simulink model "Hydrokinetic_Energy_Harvesting_Model"  (R2023a)
settings: Solver=VariableStepAuto  StartTime=0.0  StopTime=3600  RelTol=1e-3
settings Model: Creator=eeelab47  LastModifiedBy=eeelab47

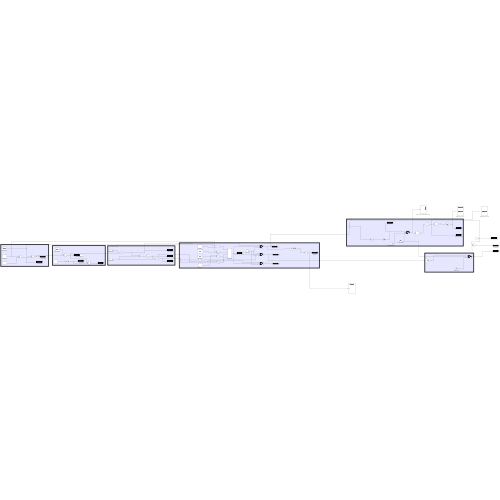
[thumbnail: Simulink's stored preview of the top-level diagram]
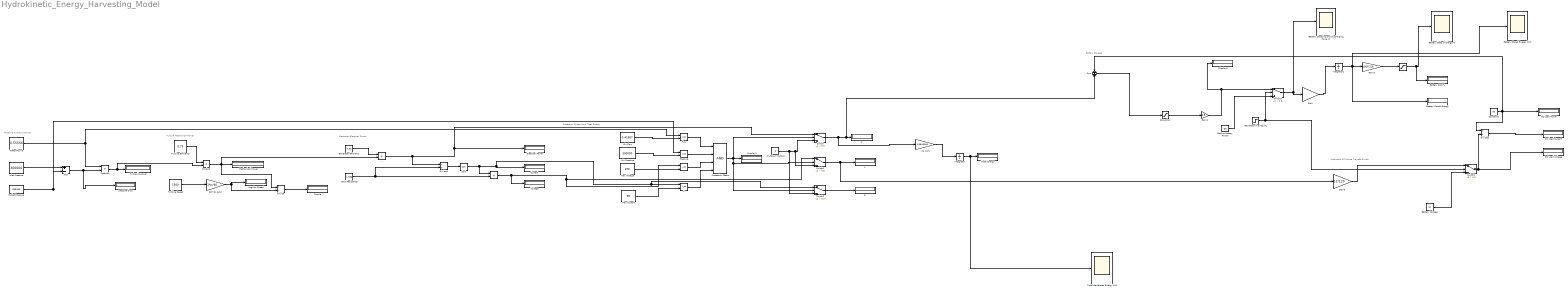
== system Hydrokinetic_Energy_Harvesting_Model ==
  note: Automatic DC Source Transfer Switch
  note: Battery Storage
  note: Protection System and Total Energy
  note: Generator Electrical Power
  note: Turbine Mechanical Power
  note: Pipeline Hydraulic Power
  " ...." : Product
  . : Saturate  UpperLimit=100  LowerLimit=0
  .. : Product
  Add : Sum  Inputs=+-
  Angular Speed : Display
  Backup Battery Power : Constant  Value=-30
  Battery Charging and Discharging Powe W : Scope
  Battery SOC % : Display
  Battery State of Charge % : Scope
  "Battery Stored Energy " : Display
  Battery Stored Energy kWh : Scope
  Battery Voltage : Constant  Value=12
  C : RelationalOperator  Operator=<=  OutDataTypeStr=boolean  RndMeth=Simplest  InputSameDT=off
  C. : Display
  Constant1 : Constant  Value=30
  Current : Display
      settings: Format=bank
  DC Load Power : Display
  DC Load Voltage : Display
  "DC load Current " : Display
  Display1 : Display
  Display5 : Display
  Divide : Product  Inputs=*/
  Divide1 : Product  Inputs=*/
  Divide2 : Product  Inputs=*/
  Electrical Power : Display
  Flow : RelationalOperator  OutDataTypeStr=boolean  RndMeth=Simplest  InputSameDT=off
  Gain : Gain  Gain=1/3600000
  Gain1 : Gain  Gain=0.9
  Gain2 : Gain  Gain=100/0.216
  Gain3 : Gain  Gain=12/120
  Generator Availability : Step  Time=1800  Before=1  After=0
  Generator Efficiency : Constant  Value=0.90
  Hydraulic power : Display
      settings: Format=bank
  Inlet Pressure : Constant  Value=360000
  Integrator : Integrator
  Integrator1 : Integrator  InitialCondition=0.108  LimitOutput=on  UpperSaturationLimit=0.216  LowerSaturationLimit=0
  J to KWh : Gain  Gain=1/3600000
  Load Resistance : Constant  Value=1.536
  Max Current : Constant  Value=90
  Max Voltage : Constant  Value=150
  Mechanical Power : Display
      settings: Format=bank
  Min Flow : Constant  Value=0.41667
  Min Pressure : Constant  Value=300000
  Outlet Pressure : Constant  Value=335000
  P. : Display
  Pressure : RelationalOperator  OutDataTypeStr=boolean  RndMeth=Simplest  InputSameDT=off
  Product : Product
  Product1 : Product
  Protection Status : Logic  Inputs=4  AllPortsSameDT=off  OutDataTypeStr=boolean
  RPM to rad/s : Gain  Gain=2*pi/60
  Saturation : Saturate  UpperLimit=43.2  LowerLimit=0
  Sqrt : Sqrt
  Sum : Sum  Inputs=-+
  Switch{,1..4} (5 alike) : Switch  Criteria=u2 > Threshold  Threshold=0.5  SaturateOnIntegerOverflow=off  InputSameDT=off
  Torque : Display
  Total Energy : Display
  Total Generated Energy kWh : Scope
  Turbine Efficiency : Constant  Value=0.75
  Turbine Speed : Constant  Value=1500
  V : RelationalOperator  Operator=<=  OutDataTypeStr=boolean  RndMeth=Simplest  InputSameDT=off
  V. : Display
  Voltage : Display
      settings: Format=bank
  Water Flow Q : Constant  Value=0.55556
  pressure Drop : Display
      settings: Format=bank
  shutdown Output : Constant  Value=0
  wires:
  Divide2/1 -> "DC load Current "/1
  Integrator/1 -> Total Generated Energy kWh/1, Total Energy/1
  Switch3/1 -> Battery Charging and Discharging Powe W/1, Gain/1
  ./1 -> Battery State of Charge %/1, Battery SOC %/1
  Integrator1/1 -> Battery Stored Energy kWh/1, "Battery Stored Energy "/1, Gain2/1
  Switch4/1 -> Divide2/2, DC Load Voltage/1
  Add/1 -> pressure Drop/1, Product1/2
  Outlet Pressure/1 -> Pressure/1, Add/2
  Divide/1 -> Torque/1
  Turbine Efficiency/1 -> Product/1
  RPM to rad/s/1 -> Angular Speed/1, Divide/2
  Product1/1 -> Product/2, Hydraulic power/1
  Turbine Speed/1 -> RPM to rad/s/1
  Product/1 -> " ...."/2, Divide/1, Mechanical Power/1
  Load Resistance/1 -> Divide1/2, ../2
  Generator Efficiency/1 -> " ...."/1
  Divide1/1 -> Sqrt/1
  " ...."/1 -> Switch/1, Electrical Power/1, Divide1/1
  Inlet Pressure/1 -> Add/1
  ../1 -> V/1, Switch1/1, Voltage/1
  V/1 -> Protection Status/3
  C/1 -> Protection Status/4
  Switch2/1 -> C./1
  Max Current/1 -> C/2
  Min Flow/1 -> Flow/2
  shutdown Output/1 -> Switch2/3, Switch1/3, Switch/3
  Flow/1 -> Protection Status/1
  Water Flow Q/1 -> Flow/1, Product1/1
  Sqrt/1 -> Switch2/1, C/1, Current/1, ../1
  Protection Status/1 -> Switch2/2, Switch1/2, Switch/2, Display1/1
  Max Voltage/1 -> V/2
  J to KWh/1 -> Integrator/1
  Pressure/1 -> Protection Status/2
  Min Pressure/1 -> Pressure/2
  Gain/1 -> Integrator1/1
  Gain2/1 -> ./1
  Constant1/1 -> Sum/1, Divide2/1, DC Load Power/1
  Switch/1 -> Sum/2, P./1, J to KWh/1
  Sum/1 -> Saturation/1
  Saturation/1 -> Gain1/1
  Gain1/1 -> Switch3/1, Display5/1
  Backup Battery Power/1 -> Switch3/3
  Switch1/1 -> Gain3/1, V./1
  Generator Availability/1 -> Switch4/2, Switch3/2
  Battery Voltage/1 -> Switch4/3
  Gain3/1 -> Switch4/1
